simulink model "Ground_Contact"  (R2026b)
settings: Solver=VariableStepAuto
undefined symbols (not defined in the file): cg_init, IN, OUT
libraries: dspmtrx3 x3, dspmathops x1, simulink x1
settings Model: Creator=asing  LastModifiedBy=asing

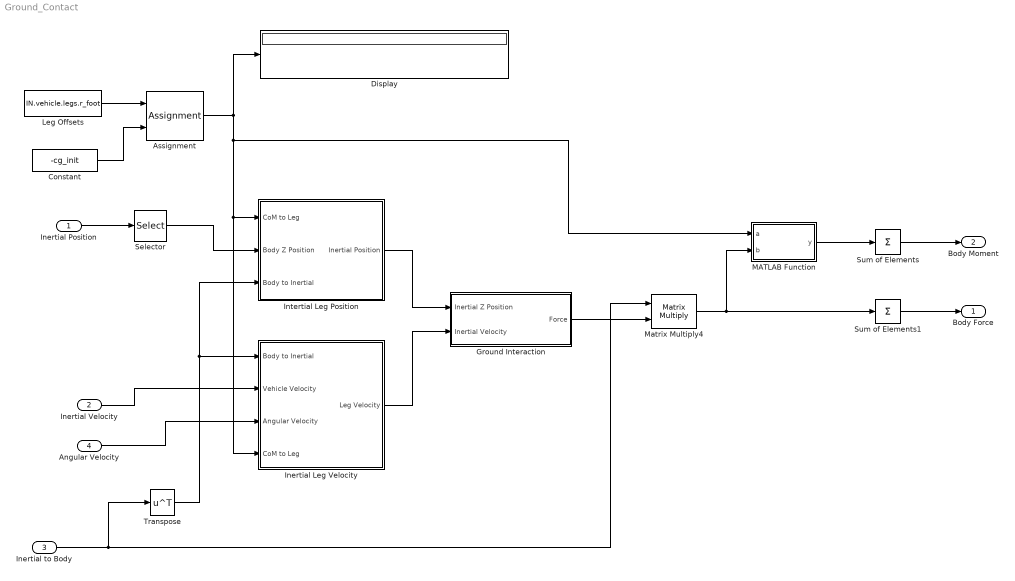
== system Ground_Contact ==
  Inertial Position : Inport
  Inertial Velocity : Inport  Port=2
  Inertial to Body : Inport  Port=3
  Angular Velocity : Inport  Port=4
  Assignment : Assignment  NumberOfDimensions=2  DiagnosticForDimensions=Warning  IndexOptions=Index vector (dialog),Assign all  Indices=1,1  OutputSizes=1,1  RuntimeRangeChecks=off
  Constant : Constant  Value=-cg_init
  Display : Display
  Ground Interaction : Subsystem
  Inertial Leg Velocity : Subsystem
  Intertial Leg Position : Subsystem
  Leg Offsets : Constant  Value=IN.vehicle.legs.r_foot
  MATLAB Function : MATLAB Function  TreatAsAtomicUnit=on
  Matrix Multiply4 : Product  Multiplication=Matrix(*)
  Selector : Selector  InputPortWidth=3  IndexOptions=Index vector (dialog)  Indices=3  OutputSizes=1  RuntimeRangeChecks=off
  Sum of Elements : Sum  Inputs=+  CollapseMode=Specified dimension  CollapseDim=2
  Sum of Elements1 : Sum  Inputs=+  CollapseMode=Specified dimension  CollapseDim=2
  Transpose : Math  Operator=transpose
  Body Force : Outport
  Body Moment : Outport  Port=2
  wires:
  Inertial to Body/1 -> Transpose/1, Matrix Multiply4/1
  Inertial Position/1 -> Selector/1
  Ground Interaction/1(Force) -> Matrix Multiply4/2
  Intertial Leg Position/1(Inertial Position) -> Ground Interaction/1(Inertial Z Position)
  Inertial Leg Velocity/1(Leg Velocity) -> Ground Interaction/2(Inertial Velocity)
  Matrix Multiply4/1 -> MATLAB Function/2(b), Sum of Elements1/1
  Selector/1 -> Intertial Leg Position/2(Body Z Position)
  Transpose/1 -> Intertial Leg Position/3(Body to Inertial), Inertial Leg Velocity/1(Body to Inertial)
  Inertial Velocity/1 -> Inertial Leg Velocity/2(Vehicle Velocity)
  Angular Velocity/1 -> Inertial Leg Velocity/3(Angular Velocity)
  Sum of Elements/1 -> Body Moment/1
  Sum of Elements1/1 -> Body Force/1
  MATLAB Function/1(y) -> Sum of Elements/1
  Assignment/1 -> MATLAB Function/1(a), Intertial Leg Position/1(CoM to Leg), Inertial Leg Velocity/4(CoM to Leg), Display/1
  Leg Offsets/1 -> Assignment/1
  Constant/1 -> Assignment/2

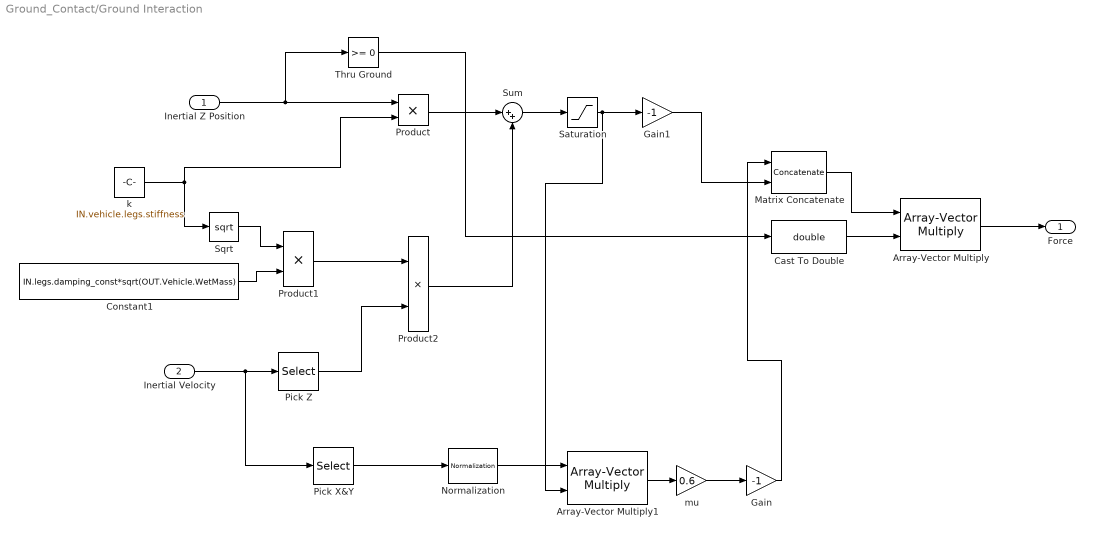
== system Ground_Contact/Ground Interaction ==
  Inertial Z Position : Inport
  Inertial Velocity : Inport  Port=2
  Array-Vector Multiply : dspmtrx3/Array-Vector Multiply  mode=Mute  saveAsFlag=0  Dimension=2  V_Source=Input port  V_VectFromMask=[0.5 0.25]  roundingMode=Floor  overflowMode=off  firstCoeffSignedness=Auto  firstCoeffDataTypeStr=Inherit: Same word length as input  firstCoeffMin=[]  firstCoeffMax=[]  firstCoeffLastDataTypeStr=Inherit: Same word length as input  prodOutputSignedness=Auto  accumSignedness=Auto  outputSignedness=Auto  outputDataTypeStr=Inherit: Same as product output  outputMin=[]  outputMax=[]  outputLastDataTypeStr=Inherit: Same as product output
  Array-Vector Multiply1 : dspmtrx3/Array-Vector Multiply  mode=Mute  saveAsFlag=0  Dimension=2  V_Source=Input port  V_VectFromMask=[0.5 0.25]  roundingMode=Floor  overflowMode=off  firstCoeffSignedness=Auto  firstCoeffDataTypeStr=Inherit: Same word length as input  firstCoeffMin=[]  firstCoeffMax=[]  firstCoeffLastDataTypeStr=Inherit: Same word length as input  prodOutputSignedness=Auto  accumSignedness=Auto  outputSignedness=Auto  outputDataTypeStr=Inherit: Same as product output  outputMin=[]  outputMax=[]  outputLastDataTypeStr=Inherit: Same as product output
  Cast To Double : DataTypeConversion  OutDataTypeStr=double  SaturateOnIntegerOverflow=off  RndMeth=Floor
  Constant1 : Constant  Value=IN.legs.damping_const*sqrt(OUT.Vehicle.WetMass)
  Gain : Gain  Gain=-1
  Gain1 : Gain  Gain=-1
  Matrix Concatenate : Concatenate  Mode=Multidimensional array
  Normalization : dspmathops/Normalization  Description=u / (|u| + IN.legs.friction_v0): Coulomb friction above v0, viscous below it (was 1e-10: full mu N in a random direction at rest)  NormType=2-norm  Bias=IN.legs.friction_v0  NormOver=Each column  Dimension=1  roundingMode=Floor  overflowMode=off  accumDataTypeStr=Inherit: Same as product output  accumLastDataTypeStr=Inherit: Same as product output  outputDataTypeStr=Inherit: Same as product output  outputMin=[]  outputMax=[]  outputLastDataTypeStr=Inherit: Same as product output
  Pick X&Y : Selector  NumberOfDimensions=2  InputPortWidth=3  IndexOptions=Index vector (dialog),Select all  Indices=[1 2],1  OutputSizes=1,1  RuntimeRangeChecks=off
  Pick Z : Selector  NumberOfDimensions=2  InputPortWidth=3  IndexOptions=Index vector (dialog),Select all  Indices=3,1  OutputSizes=1,1  RuntimeRangeChecks=off
  Product : Product
  Product1 : Product
  Product2 : Product
  Saturation : Saturate  UpperLimit=inf  LowerLimit=0
  Sqrt : Sqrt
  Sum : Sum  Inputs=|++
  Thru Ground : simulink/Logic and Bit Operations/Compare To Zero  relop=>=  OutDataTypeStr=boolean
  k : Constant  Value=IN.vehicle.legs.stiffness
  mu : Gain  Gain=0.6
  Force : Outport  OutputWhenDisabled=reset  InitialOutput=0
  wires:
  mu/1 -> Gain/1
  Array-Vector Multiply1/1 -> mu/1
  Normalization/1 -> Array-Vector Multiply1/1
  Cast To Double/1 -> Array-Vector Multiply/2
  Array-Vector Multiply/1 -> Force/1
  Matrix Concatenate/1 -> Array-Vector Multiply/1
  Thru Ground/1 -> Cast To Double/1
  Gain/1 -> Matrix Concatenate/1
  Gain1/1 -> Matrix Concatenate/2
  Pick X&Y/1 -> Normalization/1
  Saturation/1 -> Gain1/1, Array-Vector Multiply1/2
  Inertial Z Position/1 -> Product/1, Thru Ground/1
  Product2/1 -> Sum/2
  Product1/1 -> Product2/1
  Pick Z/1 -> Product2/2
  Inertial Velocity/1 -> Pick X&Y/1, Pick Z/1
  Sqrt/1 -> Product1/1
  k/1 -> Sqrt/1, Product/2
  Sum/1 -> Saturation/1
  Constant1/1 -> Product1/2
  Product/1 -> Sum/1

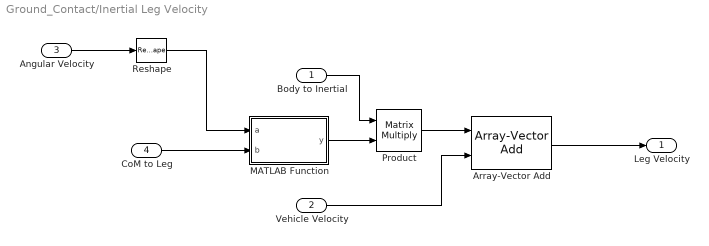
== system Ground_Contact/Inertial Leg Velocity ==
  Body to Inertial : Inport
  Vehicle Velocity : Inport  Port=2
  Angular Velocity : Inport  Port=3
  CoM to Leg : Inport  Port=4
  Array-Vector Add : dspmtrx3/Array-Vector Add  Dimension=1  V_Source=Input port  V_VectFromMask=[0.5 0.25]  prodOutputSignedness=Auto  roundingMode=Floor  overflowMode=off  firstCoeffSignedness=Auto  firstCoeffDataTypeStr=Inherit: Same word length as input  firstCoeffMin=[]  firstCoeffMax=[]  firstCoeffLastDataTypeStr=Inherit: Same word length as input  accumSignedness=Auto  outputSignedness=Auto  outputDataTypeStr=Inherit: Same as accumulator  outputMin=[]  outputMax=[]  outputLastDataTypeStr=Inherit: Same as accumulator
  MATLAB Function : MATLAB Function  TreatAsAtomicUnit=on
  Product : Product  Multiplication=Matrix(*)
  Reshape : Reshape  OutputDimensionality=Column vector (2-D)
  Leg Velocity : Outport
  wires:
  MATLAB Function/1(y) -> Product/2
  Product/1 -> Array-Vector Add/1
  CoM to Leg/1 -> MATLAB Function/2(b)
  Reshape/1 -> MATLAB Function/1(a)
  Angular Velocity/1 -> Reshape/1
  Array-Vector Add/1 -> Leg Velocity/1
  Vehicle Velocity/1 -> Array-Vector Add/2
  Body to Inertial/1 -> Product/1

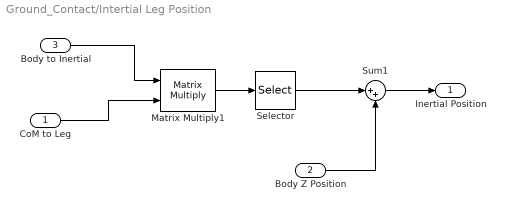
== system Ground_Contact/Intertial Leg Position ==
  CoM to Leg : Inport
  Body Z Position : Inport  Port=2
  Body to Inertial : Inport  Port=3
  Matrix Multiply1 : Product  Multiplication=Matrix(*)
  Selector : Selector  NumberOfDimensions=2  IndexOptions=Index vector (dialog),Select all  Indices=3,1  OutputSizes=1,1  RuntimeRangeChecks=off
  Sum1 : Sum  Inputs=|++
  Inertial Position : Outport
  wires:
  Selector/1 -> Sum1/1
  Sum1/1 -> Inertial Position/1
  Body to Inertial/1 -> Matrix Multiply1/1
  CoM to Leg/1 -> Matrix Multiply1/2
  Matrix Multiply1/1 -> Selector/1
  Body Z Position/1 -> Sum1/2

== matlab function Ground_Contact/MATLAB Function ==
  data: a input; y output; b input
function y = crossProduct(a, b)
    y = cross(a, b);

== matlab function Ground_Contact/Inertial Leg Velocity/MATLAB Function ==
  data: a input; y output; b input
function y = crossProduct(a, b)
    y = cross(repmat(a,1,4), b, 1);
